simulink model "MMC_phase_hackathon_circuit3_HAAS_20260216"  (R2024b)
settings: Solver=FixedStepDiscrete  StartTime=t_init_sim  StopTime=sim_time  FixedStep=Ts  RelTol=1e-3
values from neighbouring files (symbols this model uses):
  a = 1    [param_phase_circuit3_20260216.m]
  C1low1_active = 1    [script_MMC_phase_circuit3_twist_20260216.m]
  C2low1_active = 1    [script_MMC_phase_circuit3_twist_20260216.m]
  C_bus = 4400e-6    (= 0.0044)    [param_phase_circuit3_20260216.m]
  C_M_extra = C_m-twist_high_side_C    [param_phase_circuit3_20260216.m]
  duty_cycle = 0.95    [script_MMC_phase_circuit3_twist_20260216.m]
  f0 = 50    [param_phase_circuit3_20260216.m]
  feeder_current_lower_rate_limit = -10    [script_MMC_phase_circuit3_twist_20260216.m]    (also in twist_parameters.m = -500)
  feeder_current_tab = [0.328 0.217 0.162 0.132 0.109 0.094 0.083 0.075 0.068 0.062 0.058 0.054 ... (42 elements, 14x3)]    [feeder_current.mat]
  feeder_current_upper_rate_limit = 0.386/(20e-3)    (= 19.3)    [twist_parameters.m]
  is6VExternallySupplied = true    [script_MMC_phase_circuit3_twist_20260216.m]
  isFeederJumperOpen = true    [script_MMC_phase_circuit3_twist_20260216.m]
  L_arm = 60e-3    (= 0.06)    [param_phase_circuit3_20260216.m]
  m = 1    [param_phase_circuit3_20260216.m]
  N = 5    [param_phase_circuit3_20260216.m]
  power_losses = false    [script_MMC_phase_circuit3_twist_20260216.m]
  R = 15    [param_phase_circuit3_20260216.m]
  source_V = 0    [script_MMC_phase_circuit3_twist_20260216.m]
  time_charge = 0.1    [script_MMC_phase_circuit3_twist_20260216.m]
  time_decharge = 0.6    [script_MMC_phase_circuit3_twist_20260216.m]
  Ts = 5e-7    (= 5e-07)    [script_MMC_phase_circuit3_twist_20260216.m]
  twist_data_acquisition_delay = 50e-9    (= 5e-08)    [script_MMC_phase_circuit3_twist_20260216.m]    (also in twist_parameters.m)
  twist_data_sampling_period = 1/twist_freq_data_sampling    (= 5e-05)    [script_MMC_phase_circuit3_twist_20260216.m]    (also in twist_parameters.m)
  twist_dead_time = 200e-9    (= 2e-07)    [twist_parameters.m]
  twist_freq_switching = 200e3    (= 200000)    [twist_parameters.m]
  twist_high_side_adc_R = 1/(1/2e6 + 1/2e6 + 1/(330e3+5.6e3))    (= 251272.836178)    [twist_parameters.m]
  twist_high_side_C = 33e-6*4 + 4.7e-6*12    (= 0.0001884)    [twist_parameters.m]
  twist_high_side_feeder_R = 47e3+4.7e3    (= 51700)    [twist_parameters.m]
  twist_high_side_rC = 0.1    [twist_parameters.m]
  twist_low_side_adc_R = 150e3+470    (= 150470)    [twist_parameters.m]
  twist_low_side_C_ceramic = 3*4.7e-6    (= 1.41e-05)    [twist_parameters.m]
  twist_low_side_C_electrolytic = 47e-6    (= 4.7e-05)    [twist_parameters.m]
  twist_low_side_L = 33e-6    (= 3.3e-05)    [twist_parameters.m]
  twist_low_side_rC = 700e-3    (= 0.7)    [twist_parameters.m]
  twist_low_side_rL = 20e-3    (= 0.02)    [twist_parameters.m]
  twist_R_VCC = (tau_VCC/twist_high_side_C  - twist_high_side_rC)/(1-(tau_VCC/twist_high_side_C - twist_high_side_rC)/R_parallel)    (= 1110.74997822)    [twist_parameters.m]
  VDC = 48    [param_phase_circuit3_20260216.m]
undefined symbols (not defined in the file or in its folder): C_SM, feeder_current, gcbh, sps_rtmsupport, twist_low_side_lC
libraries: spsSeriesRLCBranchLib x133, spsTriangleGeneratorLib x60, spsMosfetLib x60, spsVoltageMeasurementLib x55, spsCurrentMeasurementLib x43, spsControlledCurrentSourceLib x30, spsDiodeLib x22, spsIdealSwitchLib x20, spsControlledVoltageSourceLib x1, spsGroundLib x1, spsMeanLib x1, spspowerguiLib x1
(part 7 of 18)

== system MMC_phase_hackathon_circuit3_HAAS_20260216/ /HB Twist M1/Twist Power Block/i2Low acquisition ==
  In1 : Inport
  In2 : Inport  Port=2
  If : If  IfExpression=u1 > 0.99  ShowElse=off
  If Action Subsystem : Subsystem  TreatAsAtomicUnit=on
  Scope : Scope  NumInputPorts=3
  i2Meas : Outport
  wires:
  If Action Subsystem/1(Out1) -> Scope/1, i2Meas/1  "Data_Carry"
  In1/1 -> Scope/2, If Action Subsystem/1(In1)  "Data"
  If/1 -> If Action Subsystem/Action
  In2/1 -> If/1, Scope/3  "Carry"

== system MMC_phase_hackathon_circuit3_HAAS_20260216/ /HB Twist M1/Twist Power Block/iHigh acquisition ==
  In1 : Inport
  In2 : Inport  Port=2
  If : If  IfExpression=u1 > 0.99  ShowElse=off
  If Action Subsystem : Subsystem  TreatAsAtomicUnit=on
  Scope : Scope  NumInputPorts=3
  iHMeas : Outport
  wires:
  If Action Subsystem/1(Out1) -> Scope/1, iHMeas/1  "Data_Carry"
  In1/1 -> Scope/2, If Action Subsystem/1(In1)  "Data"
  If/1 -> If Action Subsystem/Action
  In2/1 -> If/1, Scope/3  "Carry"

== system MMC_phase_hackathon_circuit3_HAAS_20260216/ /HB Twist M1/Twist Power Block/v1Low acquisition ==
  In1 : Inport
  In2 : Inport  Port=2
  If : If  IfExpression=u1 > 0.99  ShowElse=off
  If Action Subsystem : Subsystem  TreatAsAtomicUnit=on
  Scope : Scope  NumInputPorts=3
  v1Meas : Outport
  wires:
  If Action Subsystem/1(Out1) -> Scope/1, v1Meas/1  "Data_Carry"
  In1/1 -> Scope/2, If Action Subsystem/1(In1)  "Data"
  If/1 -> If Action Subsystem/Action
  In2/1 -> If/1, Scope/3  "Carry"

== system MMC_phase_hackathon_circuit3_HAAS_20260216/ /HB Twist M1/Twist Power Block/v2Low acquisition ==
  In1 : Inport
  In2 : Inport  Port=2
  If : If  IfExpression=u1 > 0.99  ShowElse=off
  If Action Subsystem : Subsystem  TreatAsAtomicUnit=on
  Scope : Scope  NumInputPorts=3
  v2Meas : Outport
  wires:
  If Action Subsystem/1(Out1) -> Scope/1, v2Meas/1  "Data_Carry"
  In1/1 -> Scope/2, If Action Subsystem/1(In1)  "Data"
  If/1 -> If Action Subsystem/Action
  In2/1 -> If/1, Scope/3  "Carry"

== system MMC_phase_hackathon_circuit3_HAAS_20260216/ /HB Twist M1/Twist Power Block/vHigh acquisition ==
  In1 : Inport
  In2 : Inport  Port=2
  If : If  IfExpression=u1 > 0.99  ShowElse=off
  If Action Subsystem : Subsystem  TreatAsAtomicUnit=on
  Scope : Scope  NumInputPorts=3
  vHMeas : Outport
  wires:
  If Action Subsystem/1(Out1) -> Scope/1, vHMeas/1  "Data_Carry"
  In1/1 -> Scope/2, If Action Subsystem/1(In1)  "Data"
  If/1 -> If Action Subsystem/Action
  In2/1 -> If/1, Scope/3  "Carry"

== system MMC_phase_hackathon_circuit3_HAAS_20260216/ /HB Twist M10/Twist Power Block/HRTimA_1 ==
  note: PWM Timer Model
  note: Note 1:
      | All sampling times inferior than Ts = 1e-6 were desactivated or changed to Ts to reduce simulation duration
  note: Note 2:
      | PWM generator original resolution value at 100 ns
  Duty cycle input : Inport
  Block : Inport  Port=2
  Constant : Constant  Value=0
  Dead Time : TransportDelay  Commented=on  DelayTime=twist_dead_time
  Demux : Demux  Outputs=2
  Logical Operator : Logic  AllPortsSameDT=off  OutDataTypeStr=boolean
  PWM Generator (2-Level) : Subsystem  AncestorBlock=|  DialogController=POWERSYS.PowerSysDialog  LoadFcn=sps_rtmsupport('LoadFcn', gcbh);  StartFcn=sps_rtmsupport('StartFcn', gcbh);  StopFcn=sps_rtmsupport('StopFcn', gcbh);  BlockChoice=InternalUref  mask(PWM Generator (2-Level)){ModulatorType=Single-phase half-bridge (2 pulses), ModulatorMode=Unsynchronized, Fc=twist_freq_switching, Pc=0, nF=27, MinMax=[0 1], SamplingTechnique=Symmetrical regular (single edge), ModulatingSignals=off, m=0.8, Freq=60, Phase=0, Ts=Ts, ShowCarrierOutport=off}
      | spsPWMGenerator2LevelLib/PWM Generator
      | (2-Level)
      mask prompts: ModulatorType "Generator type:"; ModulatorMode "Mode of operation:"; Fc "Frequency (Hz):"; Pc "Initial phase (degrees):"; nF "Switching ratio (carrier frequency / output frequency):"; MinMax "Minimum and maximum values: [ Min  Max ]"; SamplingTechnique "Sampling technique:"; ModulatingSignals "Internal generation of reference signal"; m "Modulation index:"; Freq "Frequency (Hz):"; Phase "Phase (degrees):"; Ts "Sample time (s):"; ShowCarrierOutport "Show measurement port"
      mask help:
      | Generate pulses for PWM-controlled 2-Level converter, using carrier-based two-level PWM method. The block can control switching devices of single-phase half-bridge, single-phase full-bridge (unipolar or bipolar modulation) or three-phase bridge.
      |
      | When the Synchronized mode of operation is selected, a second input is added to the block, and the internal generation of modulating signal is disabled. Use input 2 (wt) to synchronize the carrier.
      mask init:
      | sps = powericon('PWMGenerator2LevelInit',gcb,ModulatorType,SamplingTechnique,ModulatorMode,nF,Fc,MinMax,Pc,ShowCarrierOutport,ModulatingSignals,m,Freq,Phase,Ts);
      settings: CopyFcn=sps_rtmsupport('CopyFcn', gcbh);  DeleteFcn=sps_rtmsupport('DeleteFcn', gcbh);  UndoDeleteFcn=sps_rtmsupport('UndoDeleteFcn', gcbh);  ModelCloseFcn=sps_rtmsupport('ModelCloseFcn', gcbh);  PreSaveFcn=sps_rtmsupport('PreSaveFcn', gcbh);  PostSaveFcn=sps_rtmsupport('PostSaveFcn', gcbh);  NameChangeFcn=sps_rtmsupport('NameChangeFcn', gcbh);  PreCopyFcn=sps_rtmsupport('PreCopyFcn', gcbh);  OpenFcn="sps_rtmsupport('OpenFcn', gcbh, [1   2   7   8  13]);"  CloseFcn=sps_rtmsupport('CloseFcn', gcbh);  PreDeleteFcn=sps_rtmsupport('PreDeleteFcn', gcbh);
      mask Help: helpview(psbhelp);
      mask TypeOptions ModulatorType: Single-phase half-bridge (2 pulses) | Single-phase full-bridge (4 pulses) | Single-phase full-bridge - Bipolar modulation (4 pulses) | Three-phase bridge (6 pulses)
      mask TypeOptions ModulatorMode: Synchronized | Unsynchronized
      mask Callback ModulatorMode: powericon('PWMGenerator2LevelCback',gcb);
      mask TypeOptions SamplingTechnique: Natural | Asymmetrical regular (double edge) | Symmetrical regular (single edge)
      mask Callback ModulatingSignals: powericon('PWMGenerator2LevelCback',gcb);
      mask DialogControl Container3 Prompt: Carrier
      mask DialogControl ModulatingSignalParameters Prompt: Reference signal
  Peak acq : ZeroOrderHold  Commented=on  SampleTime=twist_data_acquisition_delay
  Switch : Switch  Criteria=u2 > Threshold  SaturateOnIntegerOverflow=off  InputSameDT=off
  Switch1 : Switch  Criteria=u2 > Threshold  SaturateOnIntegerOverflow=off  InputSameDT=off
  High-Side Q : Outport
  Low-Side Q : Outport  Port=2
  Carry Leg : Outport  Port=3
  wires:
  Demux/1 -> Switch/3  "high side"
  Duty cycle input/1 -> PWM Generator (2-Level)/1(Uref)  "duty_cycle"
  PWM Generator (2-Level)/2(Carry) -> Carry Leg/1, Peak acq/1  "carrier"
  Block/1 -> Switch/2, Switch1/2  "block"
  Demux/2 -> Switch1/3  "low side"
  Switch1/1 -> Low-Side Q/1
  Switch/1 -> High-Side Q/1
  Constant/1 -> Switch1/1, Switch/1
  PWM Generator (2-Level)/1(P) -> Demux/1, Dead Time/1, Logical Operator/1, Logical Operator/2  "PWM_out"

== system MMC_phase_hackathon_circuit3_HAAS_20260216/ /HB Twist M10/Twist Power Block/HRTimA_2 ==
  note: PWM Timer Model
  Duty cycle input : Inport
  Block : Inport  Port=2
  Constant : Constant  Value=0
  Dead Time : TransportDelay  Commented=on  DelayTime=twist_dead_time
  Demux : Demux  Outputs=2
  Logical Operator : Logic  AllPortsSameDT=off  OutDataTypeStr=boolean
  PWM Generator (2-Level) : Subsystem  AncestorBlock=|  DialogController=POWERSYS.PowerSysDialog  LoadFcn=sps_rtmsupport('LoadFcn', gcbh);  StartFcn=sps_rtmsupport('StartFcn', gcbh);  StopFcn=sps_rtmsupport('StopFcn', gcbh);  BlockChoice=InternalUref  mask(PWM Generator (2-Level)){ModulatorType=Single-phase half-bridge (2 pulses), ModulatorMode=Unsynchronized, Fc=twist_freq_switching, Pc=0, nF=27, MinMax=[0 1], SamplingTechnique=Symmetrical regular (single edge), ModulatingSignals=off, m=0.8, Freq=60, Phase=0, Ts=Ts, ShowCarrierOutport=off}
      | spsPWMGenerator2LevelLib/PWM Generator
      | (2-Level)
      mask prompts: ModulatorType "Generator type:"; ModulatorMode "Mode of operation:"; Fc "Frequency (Hz):"; Pc "Initial phase (degrees):"; nF "Switching ratio (carrier frequency / output frequency):"; MinMax "Minimum and maximum values: [ Min  Max ]"; SamplingTechnique "Sampling technique:"; ModulatingSignals "Internal generation of reference signal"; m "Modulation index:"; Freq "Frequency (Hz):"; Phase "Phase (degrees):"; Ts "Sample time (s):"; ShowCarrierOutport "Show measurement port"
      mask help:
      | Generate pulses for PWM-controlled 2-Level converter, using carrier-based two-level PWM method. The block can control switching devices of single-phase half-bridge, single-phase full-bridge (unipolar or bipolar modulation) or three-phase bridge.
      |
      | When the Synchronized mode of operation is selected, a second input is added to the block, and the internal generation of modulating signal is disabled. Use input 2 (wt) to synchronize the carrier.
      mask init:
      | sps = powericon('PWMGenerator2LevelInit',gcb,ModulatorType,SamplingTechnique,ModulatorMode,nF,Fc,MinMax,Pc,ShowCarrierOutport,ModulatingSignals,m,Freq,Phase,Ts);
      settings: CopyFcn=sps_rtmsupport('CopyFcn', gcbh);  DeleteFcn=sps_rtmsupport('DeleteFcn', gcbh);  UndoDeleteFcn=sps_rtmsupport('UndoDeleteFcn', gcbh);  ModelCloseFcn=sps_rtmsupport('ModelCloseFcn', gcbh);  PreSaveFcn=sps_rtmsupport('PreSaveFcn', gcbh);  PostSaveFcn=sps_rtmsupport('PostSaveFcn', gcbh);  NameChangeFcn=sps_rtmsupport('NameChangeFcn', gcbh);  PreCopyFcn=sps_rtmsupport('PreCopyFcn', gcbh);  OpenFcn="sps_rtmsupport('OpenFcn', gcbh, [1   2   7   8  13]);"  CloseFcn=sps_rtmsupport('CloseFcn', gcbh);  PreDeleteFcn=sps_rtmsupport('PreDeleteFcn', gcbh);
      mask Help: helpview(psbhelp);
      mask TypeOptions ModulatorType: Single-phase half-bridge (2 pulses) | Single-phase full-bridge (4 pulses) | Single-phase full-bridge - Bipolar modulation (4 pulses) | Three-phase bridge (6 pulses)
      mask TypeOptions ModulatorMode: Synchronized | Unsynchronized
      mask Callback ModulatorMode: powericon('PWMGenerator2LevelCback',gcb);
      mask TypeOptions SamplingTechnique: Natural | Asymmetrical regular (double edge) | Symmetrical regular (single edge)
      mask Callback ModulatingSignals: powericon('PWMGenerator2LevelCback',gcb);
      mask DialogControl Container3 Prompt: Carrier
      mask DialogControl ModulatingSignalParameters Prompt: Reference signal
  Peak acq : ZeroOrderHold  Commented=on  SampleTime=twist_data_acquisition_delay
  Switch : Switch  Criteria=u2 > Threshold  SaturateOnIntegerOverflow=off  InputSameDT=off
  Switch1 : Switch  Criteria=u2 > Threshold  SaturateOnIntegerOverflow=off  InputSameDT=off
  High-Side Q : Outport
  Low-Side Q : Outport  Port=2
  Carry Leg : Outport  Port=3
  wires:
  Logical Operator/1 -> Demux/1
  Demux/1 -> Switch/3  "high side"
  Duty cycle input/1 -> PWM Generator (2-Level)/1(Uref)  "duty_cycle"
  PWM Generator (2-Level)/2(Carry) -> Carry Leg/1, Peak acq/1  "carrier"
  Block/1 -> Switch/2, Switch1/2  "block"
  Demux/2 -> Switch1/3  "low side"
  Switch1/1 -> Low-Side Q/1
  Switch/1 -> High-Side Q/1
  Constant/1 -> Switch1/1, Switch/1
  PWM Generator (2-Level)/1(P) -> Dead Time/1, Logical Operator/1, Logical Operator/2  "PWM_out"

== system MMC_phase_hackathon_circuit3_HAAS_20260216/ /HB Twist M10/Twist Power Block/Power losses branch 1 ==
  note: Output signals
  note: Input signals
  note: Power losses calculations
  VHigh : Inport
  ILow : Inport  Port=2
  VLow : Inport  Port=3
  Add : Sum  Inputs=++++
  Branch DT loss : MATLAB Function  TreatAsAtomicUnit=on
  Branch cond loss : MATLAB Function  TreatAsAtomicUnit=on
  Branch gate loss : MATLAB Function  TreatAsAtomicUnit=on
  Branch switching loss : MATLAB Function  TreatAsAtomicUnit=on
  Divide1 : Product  Inputs=/*
  i1Loss : Outport
  wires:
  Branch switching loss/1(twist_FET_Psw) -> Add/2
  [ILow] -> Branch switching loss/2(ILow), Branch cond loss/3(ILow), Branch DT loss/1(ILow)
  Branch gate loss/1(twist_FET_Pg) -> Add/1
  Branch cond loss/1(twist_FET_Pcond) -> Add/4
  [VHigh] -> Divide1/1, Branch cond loss/1(VHigh), Branch switching loss/1(VHigh)
  Branch DT loss/1(twist_FET_Pdt) -> Add/3
  [VLow] -> Branch cond loss/2(VLow)
  Divide1/1 -> [ILoss]  "i1Loss"
  VHigh/1 -> [VHigh]
  ILow/1 -> [ILow]
  VLow/1 -> [VLow]
  [ILoss] -> i1Loss/1
  Add/1 -> Divide1/2

== system MMC_phase_hackathon_circuit3_HAAS_20260216/ /HB Twist M10/Twist Power Block/Power losses branch 2 ==
  note: Output signals
  note: Input signals
  note: Power losses calculations
  VHigh : Inport
  ILow : Inport  Port=2
  VLow : Inport  Port=3
  Add : Sum  Inputs=++++
  Branch DT loss : MATLAB Function  TreatAsAtomicUnit=on
  Branch cond loss : MATLAB Function  TreatAsAtomicUnit=on
  Branch gate loss : MATLAB Function  TreatAsAtomicUnit=on
  Branch switching loss : MATLAB Function  TreatAsAtomicUnit=on
  Divide1 : Product  Inputs=/*
  i1Loss : Outport
  wires:
  Branch switching loss/1(twist_FET_Psw) -> Add/2
  [ILow] -> Branch switching loss/2(ILow), Branch cond loss/3(ILow), Branch DT loss/1(ILow)
  Branch gate loss/1(twist_FET_Pg) -> Add/1
  Branch cond loss/1(twist_FET_Pcond) -> Add/4
  [VHigh] -> Divide1/1, Branch cond loss/1(VHigh), Branch switching loss/1(VHigh)
  Branch DT loss/1(twist_FET_Pdt) -> Add/3
  [VLow] -> Branch cond loss/2(VLow)
  Divide1/1 -> [ILoss]  "i1Loss"
  VHigh/1 -> [VHigh]
  ILow/1 -> [ILow]
  VLow/1 -> [VLow]
  [ILoss] -> i1Loss/1
  Add/1 -> Divide1/2

== system MMC_phase_hackathon_circuit3_HAAS_20260216/ /HB Twist M10/Twist Power Block/i1Low acquisition ==
  In1 : Inport
  In2 : Inport  Port=2
  If : If  IfExpression=u1 > 0.99  ShowElse=off
  If Action Subsystem : Subsystem  TreatAsAtomicUnit=on
  Scope : Scope  NumInputPorts=3
  i1Meas : Outport
  wires:
  If Action Subsystem/1(Out1) -> Scope/1, i1Meas/1  "Data_Carry"
  In1/1 -> Scope/2, If Action Subsystem/1(In1)  "Data"
  If/1 -> If Action Subsystem/Action
  In2/1 -> If/1, Scope/3  "Carry"

== system MMC_phase_hackathon_circuit3_HAAS_20260216/ /HB Twist M10/Twist Power Block/i2Low acquisition ==
  In1 : Inport
  In2 : Inport  Port=2
  If : If  IfExpression=u1 > 0.99  ShowElse=off
  If Action Subsystem : Subsystem  TreatAsAtomicUnit=on
  Scope : Scope  NumInputPorts=3
  i2Meas : Outport
  wires:
  If Action Subsystem/1(Out1) -> Scope/1, i2Meas/1  "Data_Carry"
  In1/1 -> Scope/2, If Action Subsystem/1(In1)  "Data"
  If/1 -> If Action Subsystem/Action
  In2/1 -> If/1, Scope/3  "Carry"

== system MMC_phase_hackathon_circuit3_HAAS_20260216/ /HB Twist M10/Twist Power Block/iHigh acquisition ==
  In1 : Inport
  In2 : Inport  Port=2
  If : If  IfExpression=u1 > 0.99  ShowElse=off
  If Action Subsystem : Subsystem  TreatAsAtomicUnit=on
  Scope : Scope  NumInputPorts=3
  iHMeas : Outport
  wires:
  If Action Subsystem/1(Out1) -> Scope/1, iHMeas/1  "Data_Carry"
  In1/1 -> Scope/2, If Action Subsystem/1(In1)  "Data"
  If/1 -> If Action Subsystem/Action
  In2/1 -> If/1, Scope/3  "Carry"

== system MMC_phase_hackathon_circuit3_HAAS_20260216/ /HB Twist M10/Twist Power Block/v1Low acquisition ==
  In1 : Inport
  In2 : Inport  Port=2
  If : If  IfExpression=u1 > 0.99  ShowElse=off
  If Action Subsystem : Subsystem  TreatAsAtomicUnit=on
  Scope : Scope  NumInputPorts=3
  v1Meas : Outport
  wires:
  If Action Subsystem/1(Out1) -> Scope/1, v1Meas/1  "Data_Carry"
  In1/1 -> Scope/2, If Action Subsystem/1(In1)  "Data"
  If/1 -> If Action Subsystem/Action
  In2/1 -> If/1, Scope/3  "Carry"

== system MMC_phase_hackathon_circuit3_HAAS_20260216/ /HB Twist M10/Twist Power Block/v2Low acquisition ==
  In1 : Inport
  In2 : Inport  Port=2
  If : If  IfExpression=u1 > 0.99  ShowElse=off
  If Action Subsystem : Subsystem  TreatAsAtomicUnit=on
  Scope : Scope  NumInputPorts=3
  v2Meas : Outport
  wires:
  If Action Subsystem/1(Out1) -> Scope/1, v2Meas/1  "Data_Carry"
  In1/1 -> Scope/2, If Action Subsystem/1(In1)  "Data"
  If/1 -> If Action Subsystem/Action
  In2/1 -> If/1, Scope/3  "Carry"

== system MMC_phase_hackathon_circuit3_HAAS_20260216/ /HB Twist M10/Twist Power Block/vHigh acquisition ==
  In1 : Inport
  In2 : Inport  Port=2
  If : If  IfExpression=u1 > 0.99  ShowElse=off
  If Action Subsystem : Subsystem  TreatAsAtomicUnit=on
  Scope : Scope  NumInputPorts=3
  vHMeas : Outport
  wires:
  If Action Subsystem/1(Out1) -> Scope/1, vHMeas/1  "Data_Carry"
  In1/1 -> Scope/2, If Action Subsystem/1(In1)  "Data"
  If/1 -> If Action Subsystem/Action
  In2/1 -> If/1, Scope/3  "Carry"

== system MMC_phase_hackathon_circuit3_HAAS_20260216/ /HB Twist M2/Twist Power Block/HRTimA_1 ==
  note: PWM Timer Model
  note: Note 1:
      | All sampling times inferior than Ts = 1e-6 were desactivated or changed to Ts to reduce simulation duration
  note: Note 2:
      | PWM generator original resolution value at 100 ns
  Duty cycle input : Inport
  Block : Inport  Port=2
  Constant : Constant  Value=0
  Dead Time : TransportDelay  Commented=on  DelayTime=twist_dead_time
  Demux : Demux  Outputs=2
  Logical Operator : Logic  AllPortsSameDT=off  OutDataTypeStr=boolean
  PWM Generator (2-Level) : Subsystem  AncestorBlock=|  DialogController=POWERSYS.PowerSysDialog  LoadFcn=sps_rtmsupport('LoadFcn', gcbh);  StartFcn=sps_rtmsupport('StartFcn', gcbh);  StopFcn=sps_rtmsupport('StopFcn', gcbh);  BlockChoice=InternalUref  mask(PWM Generator (2-Level)){ModulatorType=Single-phase half-bridge (2 pulses), ModulatorMode=Unsynchronized, Fc=twist_freq_switching, Pc=0, nF=27, MinMax=[0 1], SamplingTechnique=Symmetrical regular (single edge), ModulatingSignals=off, m=0.8, Freq=60, Phase=0, Ts=Ts, ShowCarrierOutport=off}
      | spsPWMGenerator2LevelLib/PWM Generator
      | (2-Level)
      mask prompts: ModulatorType "Generator type:"; ModulatorMode "Mode of operation:"; Fc "Frequency (Hz):"; Pc "Initial phase (degrees):"; nF "Switching ratio (carrier frequency / output frequency):"; MinMax "Minimum and maximum values: [ Min  Max ]"; SamplingTechnique "Sampling technique:"; ModulatingSignals "Internal generation of reference signal"; m "Modulation index:"; Freq "Frequency (Hz):"; Phase "Phase (degrees):"; Ts "Sample time (s):"; ShowCarrierOutport "Show measurement port"
      mask help:
      | Generate pulses for PWM-controlled 2-Level converter, using carrier-based two-level PWM method. The block can control switching devices of single-phase half-bridge, single-phase full-bridge (unipolar or bipolar modulation) or three-phase bridge.
      |
      | When the Synchronized mode of operation is selected, a second input is added to the block, and the internal generation of modulating signal is disabled. Use input 2 (wt) to synchronize the carrier.
      mask init:
      | sps = powericon('PWMGenerator2LevelInit',gcb,ModulatorType,SamplingTechnique,ModulatorMode,nF,Fc,MinMax,Pc,ShowCarrierOutport,ModulatingSignals,m,Freq,Phase,Ts);
      settings: CopyFcn=sps_rtmsupport('CopyFcn', gcbh);  DeleteFcn=sps_rtmsupport('DeleteFcn', gcbh);  UndoDeleteFcn=sps_rtmsupport('UndoDeleteFcn', gcbh);  ModelCloseFcn=sps_rtmsupport('ModelCloseFcn', gcbh);  PreSaveFcn=sps_rtmsupport('PreSaveFcn', gcbh);  PostSaveFcn=sps_rtmsupport('PostSaveFcn', gcbh);  NameChangeFcn=sps_rtmsupport('NameChangeFcn', gcbh);  PreCopyFcn=sps_rtmsupport('PreCopyFcn', gcbh);  OpenFcn="sps_rtmsupport('OpenFcn', gcbh, [1   2   7   8  13]);"  CloseFcn=sps_rtmsupport('CloseFcn', gcbh);  PreDeleteFcn=sps_rtmsupport('PreDeleteFcn', gcbh);
      mask Help: helpview(psbhelp);
      mask TypeOptions ModulatorType: Single-phase half-bridge (2 pulses) | Single-phase full-bridge (4 pulses) | Single-phase full-bridge - Bipolar modulation (4 pulses) | Three-phase bridge (6 pulses)
      mask TypeOptions ModulatorMode: Synchronized | Unsynchronized
      mask Callback ModulatorMode: powericon('PWMGenerator2LevelCback',gcb);
      mask TypeOptions SamplingTechnique: Natural | Asymmetrical regular (double edge) | Symmetrical regular (single edge)
      mask Callback ModulatingSignals: powericon('PWMGenerator2LevelCback',gcb);
      mask DialogControl Container3 Prompt: Carrier
      mask DialogControl ModulatingSignalParameters Prompt: Reference signal
  Peak acq : ZeroOrderHold  Commented=on  SampleTime=twist_data_acquisition_delay
  Switch : Switch  Criteria=u2 > Threshold  SaturateOnIntegerOverflow=off  InputSameDT=off
  Switch1 : Switch  Criteria=u2 > Threshold  SaturateOnIntegerOverflow=off  InputSameDT=off
  High-Side Q : Outport
  Low-Side Q : Outport  Port=2
  Carry Leg : Outport  Port=3
  wires:
  Demux/1 -> Switch/3  "high side"
  Duty cycle input/1 -> PWM Generator (2-Level)/1(Uref)  "duty_cycle"
  PWM Generator (2-Level)/2(Carry) -> Carry Leg/1, Peak acq/1  "carrier"
  Block/1 -> Switch/2, Switch1/2  "block"
  Demux/2 -> Switch1/3  "low side"
  Switch1/1 -> Low-Side Q/1
  Switch/1 -> High-Side Q/1
  Constant/1 -> Switch1/1, Switch/1
  PWM Generator (2-Level)/1(P) -> Demux/1, Dead Time/1, Logical Operator/1, Logical Operator/2  "PWM_out"

== system MMC_phase_hackathon_circuit3_HAAS_20260216/ /HB Twist M2/Twist Power Block/HRTimA_2 ==
  note: PWM Timer Model
  Duty cycle input : Inport
  Block : Inport  Port=2
  Constant : Constant  Value=0
  Dead Time : TransportDelay  Commented=on  DelayTime=twist_dead_time
  Demux : Demux  Outputs=2
  Logical Operator : Logic  AllPortsSameDT=off  OutDataTypeStr=boolean
  PWM Generator (2-Level) : Subsystem  AncestorBlock=|  DialogController=POWERSYS.PowerSysDialog  LoadFcn=sps_rtmsupport('LoadFcn', gcbh);  StartFcn=sps_rtmsupport('StartFcn', gcbh);  StopFcn=sps_rtmsupport('StopFcn', gcbh);  BlockChoice=InternalUref  mask(PWM Generator (2-Level)){ModulatorType=Single-phase half-bridge (2 pulses), ModulatorMode=Unsynchronized, Fc=twist_freq_switching, Pc=0, nF=27, MinMax=[0 1], SamplingTechnique=Symmetrical regular (single edge), ModulatingSignals=off, m=0.8, Freq=60, Phase=0, Ts=Ts, ShowCarrierOutport=off}
      | spsPWMGenerator2LevelLib/PWM Generator
      | (2-Level)
      mask prompts: ModulatorType "Generator type:"; ModulatorMode "Mode of operation:"; Fc "Frequency (Hz):"; Pc "Initial phase (degrees):"; nF "Switching ratio (carrier frequency / output frequency):"; MinMax "Minimum and maximum values: [ Min  Max ]"; SamplingTechnique "Sampling technique:"; ModulatingSignals "Internal generation of reference signal"; m "Modulation index:"; Freq "Frequency (Hz):"; Phase "Phase (degrees):"; Ts "Sample time (s):"; ShowCarrierOutport "Show measurement port"
      mask help:
      | Generate pulses for PWM-controlled 2-Level converter, using carrier-based two-level PWM method. The block can control switching devices of single-phase half-bridge, single-phase full-bridge (unipolar or bipolar modulation) or three-phase bridge.
      |
      | When the Synchronized mode of operation is selected, a second input is added to the block, and the internal generation of modulating signal is disabled. Use input 2 (wt) to synchronize the carrier.
      mask init:
      | sps = powericon('PWMGenerator2LevelInit',gcb,ModulatorType,SamplingTechnique,ModulatorMode,nF,Fc,MinMax,Pc,ShowCarrierOutport,ModulatingSignals,m,Freq,Phase,Ts);
      settings: CopyFcn=sps_rtmsupport('CopyFcn', gcbh);  DeleteFcn=sps_rtmsupport('DeleteFcn', gcbh);  UndoDeleteFcn=sps_rtmsupport('UndoDeleteFcn', gcbh);  ModelCloseFcn=sps_rtmsupport('ModelCloseFcn', gcbh);  PreSaveFcn=sps_rtmsupport('PreSaveFcn', gcbh);  PostSaveFcn=sps_rtmsupport('PostSaveFcn', gcbh);  NameChangeFcn=sps_rtmsupport('NameChangeFcn', gcbh);  PreCopyFcn=sps_rtmsupport('PreCopyFcn', gcbh);  OpenFcn="sps_rtmsupport('OpenFcn', gcbh, [1   2   7   8  13]);"  CloseFcn=sps_rtmsupport('CloseFcn', gcbh);  PreDeleteFcn=sps_rtmsupport('PreDeleteFcn', gcbh);
      mask Help: helpview(psbhelp);
      mask TypeOptions ModulatorType: Single-phase half-bridge (2 pulses) | Single-phase full-bridge (4 pulses) | Single-phase full-bridge - Bipolar modulation (4 pulses) | Three-phase bridge (6 pulses)
      mask TypeOptions ModulatorMode: Synchronized | Unsynchronized
      mask Callback ModulatorMode: powericon('PWMGenerator2LevelCback',gcb);
      mask TypeOptions SamplingTechnique: Natural | Asymmetrical regular (double edge) | Symmetrical regular (single edge)
      mask Callback ModulatingSignals: powericon('PWMGenerator2LevelCback',gcb);
      mask DialogControl Container3 Prompt: Carrier
      mask DialogControl ModulatingSignalParameters Prompt: Reference signal
  Peak acq : ZeroOrderHold  Commented=on  SampleTime=twist_data_acquisition_delay
  Switch : Switch  Criteria=u2 > Threshold  SaturateOnIntegerOverflow=off  InputSameDT=off
  Switch1 : Switch  Criteria=u2 > Threshold  SaturateOnIntegerOverflow=off  InputSameDT=off
  High-Side Q : Outport
  Low-Side Q : Outport  Port=2
  Carry Leg : Outport  Port=3
  wires:
  Logical Operator/1 -> Demux/1
  Demux/1 -> Switch/3  "high side"
  Duty cycle input/1 -> PWM Generator (2-Level)/1(Uref)  "duty_cycle"
  PWM Generator (2-Level)/2(Carry) -> Carry Leg/1, Peak acq/1  "carrier"
  Block/1 -> Switch/2, Switch1/2  "block"
  Demux/2 -> Switch1/3  "low side"
  Switch1/1 -> Low-Side Q/1
  Switch/1 -> High-Side Q/1
  Constant/1 -> Switch1/1, Switch/1
  PWM Generator (2-Level)/1(P) -> Dead Time/1, Logical Operator/1, Logical Operator/2  "PWM_out"

== system MMC_phase_hackathon_circuit3_HAAS_20260216/ /HB Twist M2/Twist Power Block/Power losses branch 1 ==
  note: Output signals
  note: Input signals
  note: Power losses calculations
  VHigh : Inport
  ILow : Inport  Port=2
  VLow : Inport  Port=3
  Add : Sum  Inputs=++++
  Branch DT loss : MATLAB Function  TreatAsAtomicUnit=on
  Branch cond loss : MATLAB Function  TreatAsAtomicUnit=on
  Branch gate loss : MATLAB Function  TreatAsAtomicUnit=on
  Branch switching loss : MATLAB Function  TreatAsAtomicUnit=on
  Divide1 : Product  Inputs=/*
  i1Loss : Outport
  wires:
  Branch switching loss/1(twist_FET_Psw) -> Add/2
  [ILow] -> Branch switching loss/2(ILow), Branch cond loss/3(ILow), Branch DT loss/1(ILow)
  Branch gate loss/1(twist_FET_Pg) -> Add/1
  Branch cond loss/1(twist_FET_Pcond) -> Add/4
  [VHigh] -> Divide1/1, Branch cond loss/1(VHigh), Branch switching loss/1(VHigh)
  Branch DT loss/1(twist_FET_Pdt) -> Add/3
  [VLow] -> Branch cond loss/2(VLow)
  Divide1/1 -> [ILoss]  "i1Loss"
  VHigh/1 -> [VHigh]
  ILow/1 -> [ILow]
  VLow/1 -> [VLow]
  [ILoss] -> i1Loss/1
  Add/1 -> Divide1/2

== system MMC_phase_hackathon_circuit3_HAAS_20260216/ /HB Twist M2/Twist Power Block/Power losses branch 2 ==
  note: Output signals
  note: Input signals
  note: Power losses calculations
  VHigh : Inport
  ILow : Inport  Port=2
  VLow : Inport  Port=3
  Add : Sum  Inputs=++++
  Branch DT loss : MATLAB Function  TreatAsAtomicUnit=on
  Branch cond loss : MATLAB Function  TreatAsAtomicUnit=on
  Branch gate loss : MATLAB Function  TreatAsAtomicUnit=on
  Branch switching loss : MATLAB Function  TreatAsAtomicUnit=on
  Divide1 : Product  Inputs=/*
  i1Loss : Outport
  wires:
  Branch switching loss/1(twist_FET_Psw) -> Add/2
  [ILow] -> Branch switching loss/2(ILow), Branch cond loss/3(ILow), Branch DT loss/1(ILow)
  Branch gate loss/1(twist_FET_Pg) -> Add/1
  Branch cond loss/1(twist_FET_Pcond) -> Add/4
  [VHigh] -> Divide1/1, Branch cond loss/1(VHigh), Branch switching loss/1(VHigh)
  Branch DT loss/1(twist_FET_Pdt) -> Add/3
  [VLow] -> Branch cond loss/2(VLow)
  Divide1/1 -> [ILoss]  "i1Loss"
  VHigh/1 -> [VHigh]
  ILow/1 -> [ILow]
  VLow/1 -> [VLow]
  [ILoss] -> i1Loss/1
  Add/1 -> Divide1/2

== system MMC_phase_hackathon_circuit3_HAAS_20260216/ /HB Twist M2/Twist Power Block/i1Low acquisition ==
  In1 : Inport
  In2 : Inport  Port=2
  If : If  IfExpression=u1 > 0.99  ShowElse=off
  If Action Subsystem : Subsystem  TreatAsAtomicUnit=on
  Scope : Scope  NumInputPorts=3
  i1Meas : Outport
  wires:
  If Action Subsystem/1(Out1) -> Scope/1, i1Meas/1  "Data_Carry"
  In1/1 -> Scope/2, If Action Subsystem/1(In1)  "Data"
  If/1 -> If Action Subsystem/Action
  In2/1 -> If/1, Scope/3  "Carry"

== system MMC_phase_hackathon_circuit3_HAAS_20260216/ /HB Twist M2/Twist Power Block/i2Low acquisition ==
  In1 : Inport
  In2 : Inport  Port=2
  If : If  IfExpression=u1 > 0.99  ShowElse=off
  If Action Subsystem : Subsystem  TreatAsAtomicUnit=on
  Scope : Scope  NumInputPorts=3
  i2Meas : Outport
  wires:
  If Action Subsystem/1(Out1) -> Scope/1, i2Meas/1  "Data_Carry"
  In1/1 -> Scope/2, If Action Subsystem/1(In1)  "Data"
  If/1 -> If Action Subsystem/Action
  In2/1 -> If/1, Scope/3  "Carry"

== system MMC_phase_hackathon_circuit3_HAAS_20260216/ /HB Twist M2/Twist Power Block/iHigh acquisition ==
  In1 : Inport
  In2 : Inport  Port=2
  If : If  IfExpression=u1 > 0.99  ShowElse=off
  If Action Subsystem : Subsystem  TreatAsAtomicUnit=on
  Scope : Scope  NumInputPorts=3
  iHMeas : Outport
  wires:
  If Action Subsystem/1(Out1) -> Scope/1, iHMeas/1  "Data_Carry"
  In1/1 -> Scope/2, If Action Subsystem/1(In1)  "Data"
  If/1 -> If Action Subsystem/Action
  In2/1 -> If/1, Scope/3  "Carry"

== system MMC_phase_hackathon_circuit3_HAAS_20260216/ /HB Twist M2/Twist Power Block/v1Low acquisition ==
  In1 : Inport
  In2 : Inport  Port=2
  If : If  IfExpression=u1 > 0.99  ShowElse=off
  If Action Subsystem : Subsystem  TreatAsAtomicUnit=on
  Scope : Scope  NumInputPorts=3
  v1Meas : Outport
  wires:
  If Action Subsystem/1(Out1) -> Scope/1, v1Meas/1  "Data_Carry"
  In1/1 -> Scope/2, If Action Subsystem/1(In1)  "Data"
  If/1 -> If Action Subsystem/Action
  In2/1 -> If/1, Scope/3  "Carry"

== system MMC_phase_hackathon_circuit3_HAAS_20260216/ /HB Twist M2/Twist Power Block/v2Low acquisition ==
  In1 : Inport
  In2 : Inport  Port=2
  If : If  IfExpression=u1 > 0.99  ShowElse=off
  If Action Subsystem : Subsystem  TreatAsAtomicUnit=on
  Scope : Scope  NumInputPorts=3
  v2Meas : Outport
  wires:
  If Action Subsystem/1(Out1) -> Scope/1, v2Meas/1  "Data_Carry"
  In1/1 -> Scope/2, If Action Subsystem/1(In1)  "Data"
  If/1 -> If Action Subsystem/Action
  In2/1 -> If/1, Scope/3  "Carry"

== system MMC_phase_hackathon_circuit3_HAAS_20260216/ /HB Twist M2/Twist Power Block/vHigh acquisition ==
  In1 : Inport
  In2 : Inport  Port=2
  If : If  IfExpression=u1 > 0.99  ShowElse=off
  If Action Subsystem : Subsystem  TreatAsAtomicUnit=on
  Scope : Scope  NumInputPorts=3
  vHMeas : Outport
  wires:
  If Action Subsystem/1(Out1) -> Scope/1, vHMeas/1  "Data_Carry"
  In1/1 -> Scope/2, If Action Subsystem/1(In1)  "Data"
  If/1 -> If Action Subsystem/Action
  In2/1 -> If/1, Scope/3  "Carry"

== system MMC_phase_hackathon_circuit3_HAAS_20260216/ /HB Twist M3/Twist Power Block/HRTimA_1 ==
  note: PWM Timer Model
  note: Note 1:
      | All sampling times inferior than Ts = 1e-6 were desactivated or changed to Ts to reduce simulation duration
  note: Note 2:
      | PWM generator original resolution value at 100 ns
  Duty cycle input : Inport
  Block : Inport  Port=2
  Constant : Constant  Value=0
  Dead Time : TransportDelay  Commented=on  DelayTime=twist_dead_time
  Demux : Demux  Outputs=2
  Logical Operator : Logic  AllPortsSameDT=off  OutDataTypeStr=boolean
  PWM Generator (2-Level) : Subsystem  AncestorBlock=|  DialogController=POWERSYS.PowerSysDialog  LoadFcn=sps_rtmsupport('LoadFcn', gcbh);  StartFcn=sps_rtmsupport('StartFcn', gcbh);  StopFcn=sps_rtmsupport('StopFcn', gcbh);  BlockChoice=InternalUref  mask(PWM Generator (2-Level)){ModulatorType=Single-phase half-bridge (2 pulses), ModulatorMode=Unsynchronized, Fc=twist_freq_switching, Pc=0, nF=27, MinMax=[0 1], SamplingTechnique=Symmetrical regular (single edge), ModulatingSignals=off, m=0.8, Freq=60, Phase=0, Ts=Ts, ShowCarrierOutport=off}
      | spsPWMGenerator2LevelLib/PWM Generator
      | (2-Level)
      mask prompts: ModulatorType "Generator type:"; ModulatorMode "Mode of operation:"; Fc "Frequency (Hz):"; Pc "Initial phase (degrees):"; nF "Switching ratio (carrier frequency / output frequency):"; MinMax "Minimum and maximum values: [ Min  Max ]"; SamplingTechnique "Sampling technique:"; ModulatingSignals "Internal generation of reference signal"; m "Modulation index:"; Freq "Frequency (Hz):"; Phase "Phase (degrees):"; Ts "Sample time (s):"; ShowCarrierOutport "Show measurement port"
      mask help:
      | Generate pulses for PWM-controlled 2-Level converter, using carrier-based two-level PWM method. The block can control switching devices of single-phase half-bridge, single-phase full-bridge (unipolar or bipolar modulation) or three-phase bridge.
      |
      | When the Synchronized mode of operation is selected, a second input is added to the block, and the internal generation of modulating signal is disabled. Use input 2 (wt) to synchronize the carrier.
      mask init:
      | sps = powericon('PWMGenerator2LevelInit',gcb,ModulatorType,SamplingTechnique,ModulatorMode,nF,Fc,MinMax,Pc,ShowCarrierOutport,ModulatingSignals,m,Freq,Phase,Ts);
      settings: CopyFcn=sps_rtmsupport('CopyFcn', gcbh);  DeleteFcn=sps_rtmsupport('DeleteFcn', gcbh);  UndoDeleteFcn=sps_rtmsupport('UndoDeleteFcn', gcbh);  ModelCloseFcn=sps_rtmsupport('ModelCloseFcn', gcbh);  PreSaveFcn=sps_rtmsupport('PreSaveFcn', gcbh);  PostSaveFcn=sps_rtmsupport('PostSaveFcn', gcbh);  NameChangeFcn=sps_rtmsupport('NameChangeFcn', gcbh);  PreCopyFcn=sps_rtmsupport('PreCopyFcn', gcbh);  OpenFcn="sps_rtmsupport('OpenFcn', gcbh, [1   2   7   8  13]);"  CloseFcn=sps_rtmsupport('CloseFcn', gcbh);  PreDeleteFcn=sps_rtmsupport('PreDeleteFcn', gcbh);
      mask Help: helpview(psbhelp);
      mask TypeOptions ModulatorType: Single-phase half-bridge (2 pulses) | Single-phase full-bridge (4 pulses) | Single-phase full-bridge - Bipolar modulation (4 pulses) | Three-phase bridge (6 pulses)
      mask TypeOptions ModulatorMode: Synchronized | Unsynchronized
      mask Callback ModulatorMode: powericon('PWMGenerator2LevelCback',gcb);
      mask TypeOptions SamplingTechnique: Natural | Asymmetrical regular (double edge) | Symmetrical regular (single edge)
      mask Callback ModulatingSignals: powericon('PWMGenerator2LevelCback',gcb);
      mask DialogControl Container3 Prompt: Carrier
      mask DialogControl ModulatingSignalParameters Prompt: Reference signal
  Peak acq : ZeroOrderHold  Commented=on  SampleTime=twist_data_acquisition_delay
  Switch : Switch  Criteria=u2 > Threshold  SaturateOnIntegerOverflow=off  InputSameDT=off
  Switch1 : Switch  Criteria=u2 > Threshold  SaturateOnIntegerOverflow=off  InputSameDT=off
  High-Side Q : Outport
  Low-Side Q : Outport  Port=2
  Carry Leg : Outport  Port=3
  wires:
  Demux/1 -> Switch/3  "high side"
  Duty cycle input/1 -> PWM Generator (2-Level)/1(Uref)  "duty_cycle"
  PWM Generator (2-Level)/2(Carry) -> Carry Leg/1, Peak acq/1  "carrier"
  Block/1 -> Switch/2, Switch1/2  "block"
  Demux/2 -> Switch1/3  "low side"
  Switch1/1 -> Low-Side Q/1
  Switch/1 -> High-Side Q/1
  Constant/1 -> Switch1/1, Switch/1
  PWM Generator (2-Level)/1(P) -> Demux/1, Dead Time/1, Logical Operator/1, Logical Operator/2  "PWM_out"

== system MMC_phase_hackathon_circuit3_HAAS_20260216/ /HB Twist M3/Twist Power Block/HRTimA_2 ==
  note: PWM Timer Model
  Duty cycle input : Inport
  Block : Inport  Port=2
  Constant : Constant  Value=0
  Dead Time : TransportDelay  Commented=on  DelayTime=twist_dead_time
  Demux : Demux  Outputs=2
  Logical Operator : Logic  AllPortsSameDT=off  OutDataTypeStr=boolean
  PWM Generator (2-Level) : Subsystem  AncestorBlock=|  DialogController=POWERSYS.PowerSysDialog  LoadFcn=sps_rtmsupport('LoadFcn', gcbh);  StartFcn=sps_rtmsupport('StartFcn', gcbh);  StopFcn=sps_rtmsupport('StopFcn', gcbh);  BlockChoice=InternalUref  mask(PWM Generator (2-Level)){ModulatorType=Single-phase half-bridge (2 pulses), ModulatorMode=Unsynchronized, Fc=twist_freq_switching, Pc=0, nF=27, MinMax=[0 1], SamplingTechnique=Symmetrical regular (single edge), ModulatingSignals=off, m=0.8, Freq=60, Phase=0, Ts=Ts, ShowCarrierOutport=off}
      | spsPWMGenerator2LevelLib/PWM Generator
      | (2-Level)
      mask prompts: ModulatorType "Generator type:"; ModulatorMode "Mode of operation:"; Fc "Frequency (Hz):"; Pc "Initial phase (degrees):"; nF "Switching ratio (carrier frequency / output frequency):"; MinMax "Minimum and maximum values: [ Min  Max ]"; SamplingTechnique "Sampling technique:"; ModulatingSignals "Internal generation of reference signal"; m "Modulation index:"; Freq "Frequency (Hz):"; Phase "Phase (degrees):"; Ts "Sample time (s):"; ShowCarrierOutport "Show measurement port"
      mask help:
      | Generate pulses for PWM-controlled 2-Level converter, using carrier-based two-level PWM method. The block can control switching devices of single-phase half-bridge, single-phase full-bridge (unipolar or bipolar modulation) or three-phase bridge.
      |
      | When the Synchronized mode of operation is selected, a second input is added to the block, and the internal generation of modulating signal is disabled. Use input 2 (wt) to synchronize the carrier.
      mask init:
      | sps = powericon('PWMGenerator2LevelInit',gcb,ModulatorType,SamplingTechnique,ModulatorMode,nF,Fc,MinMax,Pc,ShowCarrierOutport,ModulatingSignals,m,Freq,Phase,Ts);
      settings: CopyFcn=sps_rtmsupport('CopyFcn', gcbh);  DeleteFcn=sps_rtmsupport('DeleteFcn', gcbh);  UndoDeleteFcn=sps_rtmsupport('UndoDeleteFcn', gcbh);  ModelCloseFcn=sps_rtmsupport('ModelCloseFcn', gcbh);  PreSaveFcn=sps_rtmsupport('PreSaveFcn', gcbh);  PostSaveFcn=sps_rtmsupport('PostSaveFcn', gcbh);  NameChangeFcn=sps_rtmsupport('NameChangeFcn', gcbh);  PreCopyFcn=sps_rtmsupport('PreCopyFcn', gcbh);  OpenFcn="sps_rtmsupport('OpenFcn', gcbh, [1   2   7   8  13]);"  CloseFcn=sps_rtmsupport('CloseFcn', gcbh);  PreDeleteFcn=sps_rtmsupport('PreDeleteFcn', gcbh);
      mask Help: helpview(psbhelp);
      mask TypeOptions ModulatorType: Single-phase half-bridge (2 pulses) | Single-phase full-bridge (4 pulses) | Single-phase full-bridge - Bipolar modulation (4 pulses) | Three-phase bridge (6 pulses)
      mask TypeOptions ModulatorMode: Synchronized | Unsynchronized
      mask Callback ModulatorMode: powericon('PWMGenerator2LevelCback',gcb);
      mask TypeOptions SamplingTechnique: Natural | Asymmetrical regular (double edge) | Symmetrical regular (single edge)
      mask Callback ModulatingSignals: powericon('PWMGenerator2LevelCback',gcb);
      mask DialogControl Container3 Prompt: Carrier
      mask DialogControl ModulatingSignalParameters Prompt: Reference signal
  Peak acq : ZeroOrderHold  Commented=on  SampleTime=twist_data_acquisition_delay
  Switch : Switch  Criteria=u2 > Threshold  SaturateOnIntegerOverflow=off  InputSameDT=off
  Switch1 : Switch  Criteria=u2 > Threshold  SaturateOnIntegerOverflow=off  InputSameDT=off
  High-Side Q : Outport
  Low-Side Q : Outport  Port=2
  Carry Leg : Outport  Port=3
  wires:
  Logical Operator/1 -> Demux/1
  Demux/1 -> Switch/3  "high side"
  Duty cycle input/1 -> PWM Generator (2-Level)/1(Uref)  "duty_cycle"
  PWM Generator (2-Level)/2(Carry) -> Carry Leg/1, Peak acq/1  "carrier"
  Block/1 -> Switch/2, Switch1/2  "block"
  Demux/2 -> Switch1/3  "low side"
  Switch1/1 -> Low-Side Q/1
  Switch/1 -> High-Side Q/1
  Constant/1 -> Switch1/1, Switch/1
  PWM Generator (2-Level)/1(P) -> Dead Time/1, Logical Operator/1, Logical Operator/2  "PWM_out"

== system MMC_phase_hackathon_circuit3_HAAS_20260216/ /HB Twist M3/Twist Power Block/Power losses branch 1 ==
  note: Output signals
  note: Input signals
  note: Power losses calculations
  VHigh : Inport
  ILow : Inport  Port=2
  VLow : Inport  Port=3
  Add : Sum  Inputs=++++
  Branch DT loss : MATLAB Function  TreatAsAtomicUnit=on
  Branch cond loss : MATLAB Function  TreatAsAtomicUnit=on
  Branch gate loss : MATLAB Function  TreatAsAtomicUnit=on
  Branch switching loss : MATLAB Function  TreatAsAtomicUnit=on
  Divide1 : Product  Inputs=/*
  i1Loss : Outport
  wires:
  Branch switching loss/1(twist_FET_Psw) -> Add/2
  [ILow] -> Branch switching loss/2(ILow), Branch cond loss/3(ILow), Branch DT loss/1(ILow)
  Branch gate loss/1(twist_FET_Pg) -> Add/1
  Branch cond loss/1(twist_FET_Pcond) -> Add/4
  [VHigh] -> Divide1/1, Branch cond loss/1(VHigh), Branch switching loss/1(VHigh)
  Branch DT loss/1(twist_FET_Pdt) -> Add/3
  [VLow] -> Branch cond loss/2(VLow)
  Divide1/1 -> [ILoss]  "i1Loss"
  VHigh/1 -> [VHigh]
  ILow/1 -> [ILow]
  VLow/1 -> [VLow]
  [ILoss] -> i1Loss/1
  Add/1 -> Divide1/2

== system MMC_phase_hackathon_circuit3_HAAS_20260216/ /HB Twist M3/Twist Power Block/Power losses branch 2 ==
  note: Output signals
  note: Input signals
  note: Power losses calculations
  VHigh : Inport
  ILow : Inport  Port=2
  VLow : Inport  Port=3
  Add : Sum  Inputs=++++
  Branch DT loss : MATLAB Function  TreatAsAtomicUnit=on
  Branch cond loss : MATLAB Function  TreatAsAtomicUnit=on
  Branch gate loss : MATLAB Function  TreatAsAtomicUnit=on
  Branch switching loss : MATLAB Function  TreatAsAtomicUnit=on
  Divide1 : Product  Inputs=/*
  i1Loss : Outport
  wires:
  Branch switching loss/1(twist_FET_Psw) -> Add/2
  [ILow] -> Branch switching loss/2(ILow), Branch cond loss/3(ILow), Branch DT loss/1(ILow)
  Branch gate loss/1(twist_FET_Pg) -> Add/1
  Branch cond loss/1(twist_FET_Pcond) -> Add/4
  [VHigh] -> Divide1/1, Branch cond loss/1(VHigh), Branch switching loss/1(VHigh)
  Branch DT loss/1(twist_FET_Pdt) -> Add/3
  [VLow] -> Branch cond loss/2(VLow)
  Divide1/1 -> [ILoss]  "i1Loss"
  VHigh/1 -> [VHigh]
  ILow/1 -> [ILow]
  VLow/1 -> [VLow]
  [ILoss] -> i1Loss/1
  Add/1 -> Divide1/2

== system MMC_phase_hackathon_circuit3_HAAS_20260216/ /HB Twist M3/Twist Power Block/i1Low acquisition ==
  In1 : Inport
  In2 : Inport  Port=2
  If : If  IfExpression=u1 > 0.99  ShowElse=off
  If Action Subsystem : Subsystem  TreatAsAtomicUnit=on
  Scope : Scope  NumInputPorts=3
  i1Meas : Outport
  wires:
  If Action Subsystem/1(Out1) -> Scope/1, i1Meas/1  "Data_Carry"
  In1/1 -> Scope/2, If Action Subsystem/1(In1)  "Data"
  If/1 -> If Action Subsystem/Action
  In2/1 -> If/1, Scope/3  "Carry"

== system MMC_phase_hackathon_circuit3_HAAS_20260216/ /HB Twist M3/Twist Power Block/i2Low acquisition ==
  In1 : Inport
  In2 : Inport  Port=2
  If : If  IfExpression=u1 > 0.99  ShowElse=off
  If Action Subsystem : Subsystem  TreatAsAtomicUnit=on
  Scope : Scope  NumInputPorts=3
  i2Meas : Outport
  wires:
  If Action Subsystem/1(Out1) -> Scope/1, i2Meas/1  "Data_Carry"
  In1/1 -> Scope/2, If Action Subsystem/1(In1)  "Data"
  If/1 -> If Action Subsystem/Action
  In2/1 -> If/1, Scope/3  "Carry"

== system MMC_phase_hackathon_circuit3_HAAS_20260216/ /HB Twist M3/Twist Power Block/iHigh acquisition ==
  In1 : Inport
  In2 : Inport  Port=2
  If : If  IfExpression=u1 > 0.99  ShowElse=off
  If Action Subsystem : Subsystem  TreatAsAtomicUnit=on
  Scope : Scope  NumInputPorts=3
  iHMeas : Outport
  wires:
  If Action Subsystem/1(Out1) -> Scope/1, iHMeas/1  "Data_Carry"
  In1/1 -> Scope/2, If Action Subsystem/1(In1)  "Data"
  If/1 -> If Action Subsystem/Action
  In2/1 -> If/1, Scope/3  "Carry"

== system MMC_phase_hackathon_circuit3_HAAS_20260216/ /HB Twist M3/Twist Power Block/v1Low acquisition ==
  In1 : Inport
  In2 : Inport  Port=2
  If : If  IfExpression=u1 > 0.99  ShowElse=off
  If Action Subsystem : Subsystem  TreatAsAtomicUnit=on
  Scope : Scope  NumInputPorts=3
  v1Meas : Outport
  wires:
  If Action Subsystem/1(Out1) -> Scope/1, v1Meas/1  "Data_Carry"
  In1/1 -> Scope/2, If Action Subsystem/1(In1)  "Data"
  If/1 -> If Action Subsystem/Action
  In2/1 -> If/1, Scope/3  "Carry"

== system MMC_phase_hackathon_circuit3_HAAS_20260216/ /HB Twist M3/Twist Power Block/v2Low acquisition ==
  In1 : Inport
  In2 : Inport  Port=2
  If : If  IfExpression=u1 > 0.99  ShowElse=off
  If Action Subsystem : Subsystem  TreatAsAtomicUnit=on
  Scope : Scope  NumInputPorts=3
  v2Meas : Outport
  wires:
  If Action Subsystem/1(Out1) -> Scope/1, v2Meas/1  "Data_Carry"
  In1/1 -> Scope/2, If Action Subsystem/1(In1)  "Data"
  If/1 -> If Action Subsystem/Action
  In2/1 -> If/1, Scope/3  "Carry"

== system MMC_phase_hackathon_circuit3_HAAS_20260216/ /HB Twist M3/Twist Power Block/vHigh acquisition ==
  In1 : Inport
  In2 : Inport  Port=2
  If : If  IfExpression=u1 > 0.99  ShowElse=off
  If Action Subsystem : Subsystem  TreatAsAtomicUnit=on
  Scope : Scope  NumInputPorts=3
  vHMeas : Outport
  wires:
  If Action Subsystem/1(Out1) -> Scope/1, vHMeas/1  "Data_Carry"
  In1/1 -> Scope/2, If Action Subsystem/1(In1)  "Data"
  If/1 -> If Action Subsystem/Action
  In2/1 -> If/1, Scope/3  "Carry"
